simulink model "Pack_Grouped"  (R2026b)
settings: Solver=VariableStepAuto
undefined symbols (not defined in the file or in its folder): P, Ts
libraries: nesl_utility x1, Shaddad_Battery_lib x1
settings Model: Creator=aomar  LastModifiedBy=aomar

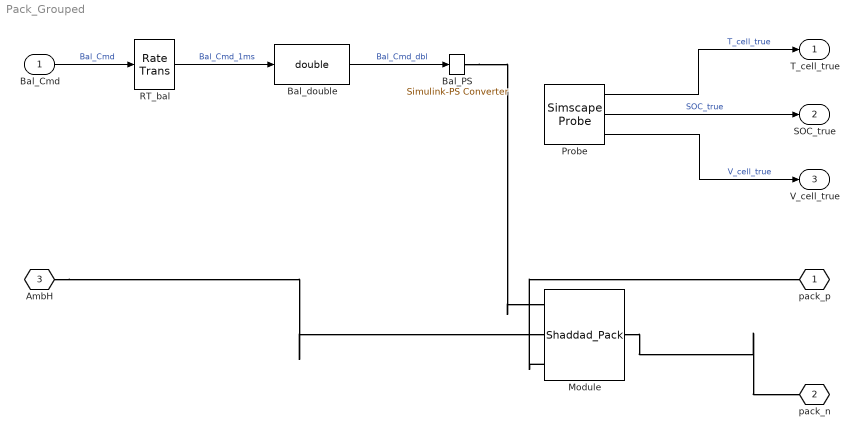
== system Pack_Grouped ==
  Bal_Cmd : Inport  OutDataTypeStr=boolean  PortDimensions=P.power.pack.Ns  SampleTime=Ts.bms_fast
  Bal_PS : nesl_utility/Simulink-PS Converter  PhysicalDomain=network_engine_domain  SubClassName=ps_input  LeftPortType=input  RightPortType=output  PseudoPeriodic=off  Frequencies=[]  NoiseDistribution=none  NoiseParameters=[]  Unit=1  AffineConversion=off  FilteringAndDerivatives=zero  SimscapeFilterOrder=1  InputFilterTimeConstant=0.001  UdotUserProvided=0
  Bal_double : DataTypeConversion  OutDataTypeStr=double  SaturateOnIntegerOverflow=off  RndMeth=Floor
  Module : Shaddad_Battery_lib/Shaddad_Pack  BatteryCapacityCell=P.power.cell.Q_Ah*P.power.pack.age.cap_factor A*hr  BatteryCapacityCellPercentDeviation=P.power.pack.var.cap_dev_pct(:)  ExtrapolationMethodCell=simscape.enum.extrapolation.linear  SOCBreakpointsCell=P.power.cell.SOC_bp  SOCBreakpointsCellPercentDeviation=zeros(P.power.pack.Ns,1)  TemperatureBreakpointsCell=P.power.cell.T_bp K  TemperatureBreakpointsCellPercentDeviation=zeros(P.power.pack.Ns,1)  OpenCircuitVoltageThermalCell=P.power.cell.OCV_tab V  OpenCircuitVoltageThermalCellPercentDeviation=zeros(P.power.pack.Ns,1)  VoltageRangeCell=P.power.cell.VoltageRange V  VoltageRangeCellPercentDeviation=zeros(P.power.pack.Ns,1)  ResistanceSOCBreakpointsCell=P.power.cell.SOC_bp  ResistanceSOCBreakpointsCellPercentDeviation=zeros(P.power.pack.Ns,1)  ResistanceTemperatureBreakpointsCell=P.power.cell.T_bp K  ResistanceTemperatureBreakpointsCellPercentDeviation=zeros(P.power.pack.Ns,1)  R0ThermalCell=P.power.cell.R0_tab*P.power.pack.age.R0_factor Ohm  R0ThermalCellPercentDeviation=P.power.pack.var.R0_dev_pct(:)  R1ThermalCell=P.power.cell.R1_tab Ohm  R1ThermalCellPercentDeviation=zeros(P.power.pack.Ns,1)  Tau1ThermalCell=P.power.cell.tau1_tab s  Tau1ThermalCellPercentDeviation=zeros(P.power.pack.Ns,1)  BatteryThermalMassCell=P.power.cell.Cth J/K  BatteryThermalMassCellPercentDeviation=zeros(P.power.pack.Ns,1)  AmbientResistance=P.power.pack.R_amb_cell K/W  NonCellElectricalResistance=P.power.pack.R_noncell_total Ohm  CellBalancingClosedResistance=P.power.pack.bal_Rsw_cell Ohm  CellBalancingOpenConductance=P.power.pack.bal_G_open 1/Ohm  CellBalancingThreshold=P.power.pack.bal_threshold  CellBalancingResistance=P.power.pack.bal_R_cell Ohm  socCell_specify=on  socCell_priority=High  socCell=P.power.pack.var.SOC0_vec(:)  socCell_nominal_specify=off  socCell_nominal_value=1  socCell_nominal_unit=1  batteryVoltage_specify=off  batteryVoltage_priority=None  batteryVoltage=repmat(0, 13, 1) V  batteryVoltage_nominal_specify=off  batteryVoltage_nominal_value=1  batteryVoltage_nominal_unit=V  batteryCurrent_specify=off  batteryCurrent_priority=None  batteryCurrent=repmat(0, 13, 1) A  batteryCurrent_nominal_specify=off  batteryCurrent_nominal_value=1  batteryCurrent_nominal_unit=A  numCycles_specify=off  numCycles_priority=High  numCycles=repmat(0, 13, 1)  numCycles_nominal_specify=off  numCycles_nominal_value=1  numCycles_nominal_unit=1  batteryTemperature_specify=on  batteryTemperature_priority=High  batteryTemperature=P.power.thermal.T_init_K*ones(P.power.pack.Ns,1) K  batteryTemperature_nominal_specify=off  batteryTemperature_nominal_value=1  batteryTemperature_nominal_unit=K  vParallelAssembly_specify=off  vParallelAssembly_priority=None  vParallelAssembly=repmat(0, 13, 1) V  vParallelAssembly_nominal_specify=off  vParallelAssembly_nominal_value=1  vParallelAssembly_nominal_unit=V  socParallelAssembly_specify=off  socParallelAssembly_priority=None  socParallelAssembly=repmat(1, 13, 1)  socParallelAssembly_nominal_specify=off  socParallelAssembly_nominal_value=1  socParallelAssembly_nominal_unit=1
  Probe : SimscapeProbe  BoundBlock=8  Variables="{\"batteryTemperature\":{\"Probing\":\"ON\"},\"socParallelAssembly\":{\"Probing\":\"ON\"},\"vParallelAssembly\":{\"Probing\":\"ON\"}}"
  RT_bal : RateTransition  OutPortSampleTime=Ts.base
  pack_p : PMIOPort  Side=Right  ConnectionType=Connection: foundation.electrical.electrical
  pack_n : PMIOPort  Port=2  Side=Right  ConnectionType=Connection: foundation.electrical.electrical
  AmbH : PMIOPort  Port=3  Side=Left  ConnectionType=Connection: foundation.thermal.thermal
  T_cell_true : Outport  OutDataTypeStr=double
  SOC_true : Outport  Port=2  OutDataTypeStr=double
  V_cell_true : Outport  Port=3  OutDataTypeStr=double
  wires:
  Bal_Cmd/1 -> RT_bal/1  "Bal_Cmd"
  RT_bal/1 -> Bal_double/1  "Bal_Cmd_1ms"
  Bal_double/1 -> Bal_PS/1  "Bal_Cmd_dbl"
  Probe/1 -> T_cell_true/1  "T_cell_true"
  Probe/2 -> SOC_true/1  "SOC_true"
  Probe/3 -> V_cell_true/1  "V_cell_true"
  connections:
  AmbH/RConn1 -- Module/LConn2
  Bal_PS/RConn1 -- Module/LConn1
  Module/LConn3 -- pack_p/RConn1
  Module/RConn1 -- pack_n/RConn1
